simulink model "hrg_wa_v10_2_cn_port_bench"  (R2025a)
settings: Solver=FixedStepDiscrete  StartTime=0.0  StopTime=p.duration  FixedStep=p.Ts  RelTol=1e-3
model workspace (MAT data in the model file):
  Ad = [0.987688405123 5.68131323296e-08 -982.899001209 0.00680633562581 0 0 943869.866875 -6.2854468604 113668107.931 -505.246320907 62170953.3395 -882829.706009 ... (144 elements, 12x12)]
  Bd = [1.07541978092e-16 2.15044631223e-18 1.17750014529e-11 2.35440509738e-13 0.71349520314 0 -1.10105605369e-08 -2.20157780066e-10 -9.65252715165e-07 -1.93016562843e-08 -4.58609339763e-07 -2.49830556256e-09 ... (24 elements, 12x2)]
  bench_input = [0 2.5e-05 5e-05 7.5e-05 0.0001 0.000125 0.00015 0.000175 0.0002 0.000225 0.00025 0.000275 ... (3603 elements, 1201x3)]
  c : object (value not decoded)
  p : object (value not decoded)
  x0 = [2.76318298201e-12; 1.16825502693e-12; 0; 0; 0; 0; 0; 0; 0; 0; 0; 0]
symbols that are objects in the model workspace (value not decoded): p
libraries: hrg_wa_v10_2_cn_modules x5
(part 2 of 2)

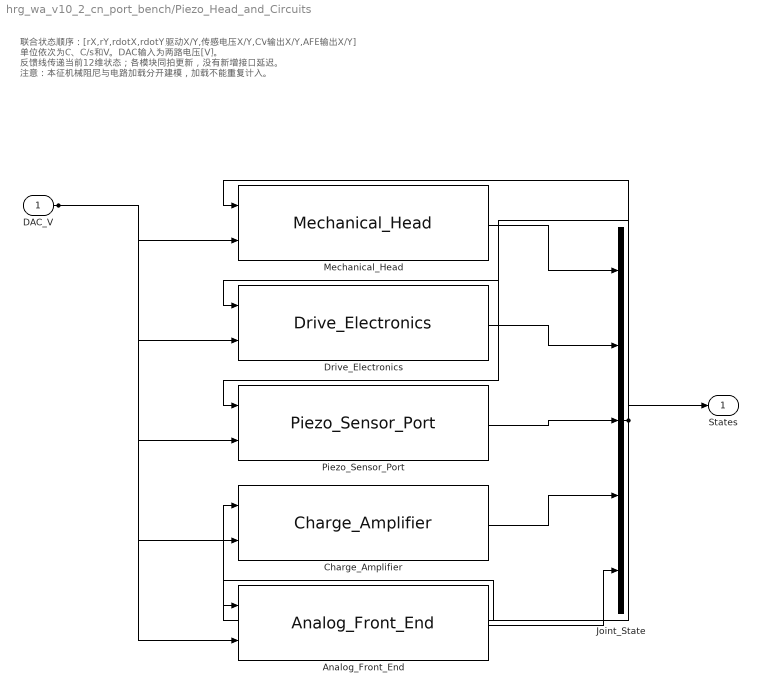
== system hrg_wa_v10_2_cn_port_bench/Piezo_Head_and_Circuits ==
  note: 联合状态顺序：[rX,rY,rdotX,rdotY,驱动X/Y,传感电压X/Y,CV输出X/Y,AFE输出X/Y]
      | 单位依次为C、C/s和V。DAC输入为两路电压[V]。
      | 反馈线传递当前12维状态；各模块同拍更新，没有新增接口延迟。
      | 注意：本征机械阻尼与电路加载分开建模，加载不能重复计入。
  DAC_V : Inport
  Analog_Front_End : hrg_wa_v10_2_cn_modules/Analog_Front_End  Description=|  SystemSampleTime=-1  VariantActivationTime=update diagram  EmptyChoice=off  PassThrough=off  PassThroughVariantControl=(default)  EmptyChoiceVariantControl=(default)  AllowFlexibleInterface=on  Latency=0  AutoFrameSizeCalculation=off
      | 模拟前端AFE｜带宽及通道耦合
      | 状态11:12为ADC前电压[V]。afe_bw为Hz，内部乘2π换成角频率。
      | 检测矩阵包含两通道幅值不一致与串扰。
  Charge_Amplifier : hrg_wa_v10_2_cn_modules/Charge_Amplifier  Description=|  SystemSampleTime=-1  VariantActivationTime=update diagram  EmptyChoice=off  PassThrough=off  PassThroughVariantControl=(default)  EmptyChoiceVariantControl=(default)  AllowFlexibleInterface=on  Latency=0  AutoFrameSizeCalculation=off
      | 电荷放大器｜积分及泄放
      | 状态9:10为输出电压[V]。Cf决定电荷/电压增益，Rf提供直流泄放。
      | 输出还需经过AFE，不能直接当作理想运动电荷。
  Drive_Electronics : hrg_wa_v10_2_cn_modules/Drive_Electronics  Description=|  SystemSampleTime=-1  VariantActivationTime=update diagram  EmptyChoice=off  PassThrough=off  PassThroughVariantControl=(default)  EmptyChoiceVariantControl=(default)  AllowFlexibleInterface=on  Latency=0  AutoFrameSizeCalculation=off
      | 驱动电子学｜双通道一阶带宽
      | 状态5:6为驱动器电压[V]。DAC输入为两路采样电压[V]。
      | 通道时间常数driver_tau及drive_matrix描述不一致与串扰。
  Joint_State : Mux  Inputs=5
  Mechanical_Head : hrg_wa_v10_2_cn_modules/Mechanical_Head  Description=|  SystemSampleTime=-1  VariantActivationTime=update diagram  EmptyChoice=off  PassThrough=off  PassThroughVariantControl=(default)  EmptyChoiceVariantControl=(default)  AllowFlexibleInterface=on  Latency=0  AutoFrameSizeCalculation=off
      | 机械表头｜二维二阶模态
      | 状态1:2为运动电荷r[C]，3:4为电荷速度[C/s]。
      | 刚度、阻尼可有不同主轴；角速度经科里奥利项耦合。
      | 输入是当前联合12维状态和DAC电压，不是独立机械力接口。
  Piezo_Sensor_Port : hrg_wa_v10_2_cn_modules/Piezo_Sensor_Port  Description=|  SystemSampleTime=-1  VariantActivationTime=update diagram  EmptyChoice=off  PassThrough=off  PassThroughVariantControl=(default)  EmptyChoiceVariantControl=(default)  AllowFlexibleInterface=on  Latency=0  AutoFrameSizeCalculation=off
      | 压电传感端口｜互易机电加载
      | 状态7:8为节点电压[V]。Cs、G0、Rs及运动电荷电流共同作用。
      | 端口电压回作用机械运动；不可把加载衰减率再次加到本征阻尼。
  States : Outport
  wires:
  Joint_State/1 -> Mechanical_Head/1, Drive_Electronics/1, Piezo_Sensor_Port/1, Charge_Amplifier/1, Analog_Front_End/1, States/1
  DAC_V/1 -> Mechanical_Head/2, Drive_Electronics/2, Piezo_Sensor_Port/2, Charge_Amplifier/2, Analog_Front_End/2
  Mechanical_Head/1 -> Joint_State/1
  Drive_Electronics/1 -> Joint_State/2
  Piezo_Sensor_Port/1 -> Joint_State/3
  Charge_Amplifier/1 -> Joint_State/4
  Analog_Front_End/1 -> Joint_State/5
